simulink model "intr"  (R2024b)
settings: Solver=VariableStepAuto  StartTime=0.0  StopTime=20.0  RelTol=1e-3
model workspace (MAT data in the model file):
  x1 = 1
  y1 = 1
  y2 = 2
settings Model: Creator=rober  LastModifiedBy=rober

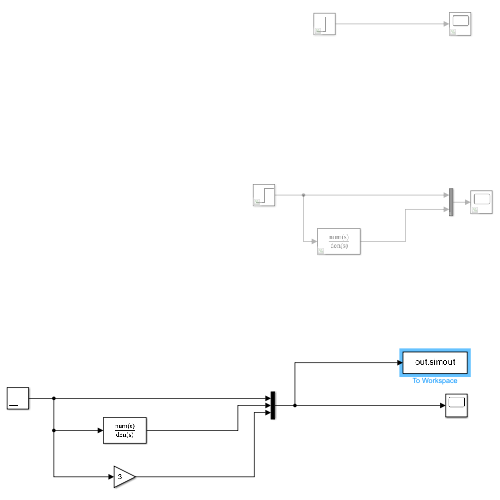
[thumbnail: Simulink's stored preview of the top-level diagram]
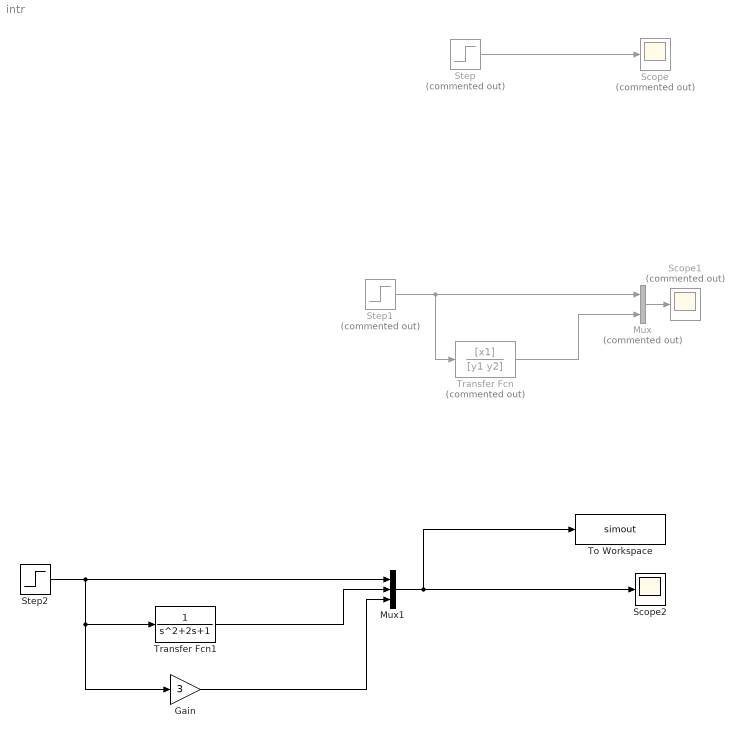
== system intr ==
  Gain : Gain  Gain=3
  Mux : Mux  Commented=on  Inputs=2
  Mux1 : Mux  Inputs=3
  Scope : Scope  Commented=on
  Scope1 : Scope  Commented=on
  Scope2 : Scope
  Step : Step  Commented=on  SampleTime=0
  Step1 : Step  Commented=on  SampleTime=0
  Step2 : Step  Time=5  Before=2  After=4  SampleTime=0
  To Workspace : ToWorkspace  VariableName=simout  SaveFormat=Timeseries  SampleTime=-1
  Transfer Fcn : TransferFcn  Commented=on  Numerator=[x1]  Denominator=[y1 y2]
  Transfer Fcn1 : TransferFcn
  wires:
  Step/1 -> Scope/1
  Mux/1 -> Scope1/1
  Transfer Fcn/1 -> Mux/2
  Step1/1 -> Transfer Fcn/1, Mux/1
  Step2/1 -> Transfer Fcn1/1, Gain/1, Mux1/1
  Mux1/1 -> Scope2/1, To Workspace/1
  Transfer Fcn1/1 -> Mux1/2
  Gain/1 -> Mux1/3
